simulink model "dual_thyristor_bridge_rectifier"  (R2025b)
settings: Solver=ode1be  StartTime=0.0  StopTime=simlength  FixedStep=tc  MaxStep=tc
values from neighbouring files (symbols this model uses):
  n1 = 35    [voltage_spectrum_analysis.m]
  omega_grid_emulator_nom = w_grid    (= 314.159265359)    [grid_emulator.m]
  vn_eta_pu = 0    [grid_emulator.m]
  vn_xi_pu = 0    [grid_emulator.m]
  vp_xi_pu = 1    [grid_emulator.m]
  w_grid = f_grid*2*pi    (= 314.159265359)    [grid_emulator.m]
undefined symbols (not defined in the file or in its folder): CSF_11, CSF_13, CSF_5, CSF_7, delta_fht1, Idc_traction_normalization_factor, ki_u_ctrl, kp_u_ctrl, Ld_fht1, LFu_dc, LSF_11, LSF_13, LSF_5, LSF_7, magnitude, n10, omega_fht1, pll_i1, pll_p, RLFu_dc, tc, Tcontrol_rect, ts_ctrl_rect, ugrid_factor, Vdc_traction_normalization_factor, Vgrid_phase_normalization_factor
libraries: fl_lib x299, nesl_utility x67, ee_lib x24, single_phase_transformer_lib x3, cstblocks x3
(part 5 of 6)

== system dual_thyristor_bridge_rectifier/dual_rectifier_bridge/pos_bridge/firing4 ==
  Capacitor1 : fl_lib/Electrical/Electrical Elements/Capacitor  Commented=on  c=100e-6 F  r=1e-6 Ohm  g=0 1/Ohm  i_specify=off  i_priority=None  i=0 A  i_nominal_specify=off  i_nominal_value=1  i_nominal_unit=A  v_specify=off  v_priority=None  v=0 V  v_nominal_specify=off  v_nominal_value=1  v_nominal_unit=V  vc_specify=off  vc_priority=High  vc=0 V  vc_nominal_specify=off  vc_nominal_value=1  vc_nominal_unit=V
  Capacitor2 : fl_lib/Electrical/Electrical Elements/Capacitor  Commented=on  c=100e-12 F  r=1e-6 Ohm  g=0 1/Ohm  i_specify=off  i_priority=None  i=0 A  i_nominal_specify=off  i_nominal_value=1  i_nominal_unit=A  v_specify=off  v_priority=None  v=0 V  v_nominal_specify=off  v_nominal_value=1  v_nominal_unit=V  vc_specify=off  vc_priority=High  vc=0 V  vc_nominal_specify=off  vc_nominal_value=1  vc_nominal_unit=V
  Controlled Voltage Source1 : fl_lib/Electrical/Electrical Sources/Controlled Voltage Source  Commented=on
  Controlled Voltage Source2 : fl_lib/Electrical/Electrical Sources/Controlled Voltage Source  Commented=on
  Diode : fl_lib/Electrical/Electrical Elements/Diode  Commented=on  Vf=0.6 V  Ron=0.3 Ohm  Goff=1e-8 1/Ohm  i_specify=off  i_priority=None  i=0 A  i_nominal_specify=off  i_nominal_value=1  i_nominal_unit=A  v_specify=off  v_priority=None  v=0 V  v_nominal_specify=off  v_nominal_value=1  v_nominal_unit=V
  Diode2 : fl_lib/Electrical/Electrical Elements/Diode  Commented=on  Vf=0.6 V  Ron=0.3 Ohm  Goff=1e-8 1/Ohm  i_specify=off  i_priority=None  i=0 A  i_nominal_specify=off  i_nominal_value=1  i_nominal_unit=A  v_specify=off  v_priority=None  v=0 V  v_nominal_specify=off  v_nominal_value=1  v_nominal_unit=V
  Diode3 : fl_lib/Electrical/Electrical Elements/Diode  Commented=on  Vf=0.6 V  Ron=0.3 Ohm  Goff=1e-8 1/Ohm  i_specify=off  i_priority=None  i=0 A  i_nominal_specify=off  i_nominal_value=1  i_nominal_unit=A  v_specify=off  v_priority=None  v=0 V  v_nominal_specify=off  v_nominal_value=1  v_nominal_unit=V
  Electrical Reference3 : fl_lib/Electrical/Electrical Elements/Electrical Reference  Commented=on
  Electrical Reference4 : fl_lib/Electrical/Electrical Elements/Electrical Reference  Commented=on
  Electrical Reference5 : fl_lib/Electrical/Electrical Elements/Electrical Reference  Commented=on
  "IGBT (Ideal, Switching)" : ee_lib/Semiconductors & Converters/IGBT (Ideal, Switching)  Commented=on  port_option=ee.enum.controlport.elec  Vf=0.8 V  Ron=0.001 Ohm  Goff=1e-5 1/Ohm  Vth=2 V  diode_param=1  diode_Vf=0.8 V  diode_Ron=0.001 Ohm  diode_Goff=1e-5 1/Ohm  diode_C=50e-9 F  diode_iRM=-235 A  diode_iF=300 A  diode_idot=-50 A/us  diode_trr_param=1  diode_trr_factor=3  diode_trr=15 us  diode_Qrr=1500 s*uA  ice_specify=off  ice_priority=None  ice=0 A  ice_nominal_specify=off  ice_nominal_value=1  ice_nominal_unit=A  vce_specify=off  vce_priority=None  vce=0 V  vce_nominal_specify=off  vce_nominal_value=1  vce_nominal_unit=V  vge_specify=off  vge_priority=None  vge=0 V  vge_nominal_specify=off  vge_nominal_value=1  vge_nominal_unit=V  thermal_loss_option=2  Von_data=[0, 1.1, 1.3, 1.45, 1.75, 2.25, 2.7; 0, 1, 1.15, 1.35, 1.7, 2.35, 3] V  Tj=[298.15, 398.15] K  Iout_data=[0, 10, 50, 100, 200, 400, 600] A  Eon_data=[0, .29, 1.43, 2.86, 5.71, 13.14, 22.86; 0, .57, 2.63, 5.14, 10.29, 20.57, 30.29] * 1e-3 J  Eoff_data=[0, .21, 1.07, 2.14, 4.29, 9.86, 17.14; 0, .43, 1.97, 3.86, 7.71, 15.43, 22.71] * 1e-3 J  Eon_data_3D=[zeros(2, 9, 3)] J  Eoff_data_3D=[zeros(2, 9, 3)] J  Tj_loss=[298.15, 398.15] K  Iout_data_loss=[0, .1, 1, 5, 10, 20, 40, 70, 100] A  tabulateWithVce=false  Vce_loss=[0, 150, 300] V  Eon_scalar=22.86e-3 J  Eoff_scalar=17.14e-3 J  Voff=300 V  Iout_scalar=600 A  useCurrentFromPreviousCycle=false  useVoltageFromPreviousCycle=false  diodeModelType=ee.enum.converters.diodeModelType.pwl  diodeTableType=ee.enum.diode.tableType.IfMat  diode_ReverseIVType=ee.enum.diode.diodeReverseIV.constant  diode_IfMat=[.07, .12, .19, 1.75, 4.24, 7.32, 11.2; .16, .3, .72, 2.14, 4.02, 6.35, 9.12] A  diode_VfMat=[.9, 1.15, 1.25, 1.5, 1.75, 2.17, 2.6, 2.85; .58, .68, .75, 1.1, 1.38, 1.77, 2.27, 2.7] V  diode_TjVec=[25, 125] degC  diode_VfVec=[.5, .7, .9, 1.3, 1.7, 2.1, 2.5] V  diode_IfVec=[.1, .2, .5, 1, 2, 4, 7, 10] A  diode_IrMat=[1e-06, 2e-06, 5e-06, 1e-05, 2.5e-05, 5e-05, .0001; 2e-06, 5e-06, 1e-05, 4e-05, 8e-05, .0002, .0005] A  diode_VrMat=[10, 100, 200, 250, 300, 325, 350; 10, 70, 160, 220, 270, 300, 320] V  diode_VrVec=[10, 20, 40, 50, 70, 80, 100] V  diode_IrVec=[1e-06, 2e-06, 5e-06, 1e-05, 2e-05, 5e-05, .0001] A  diode_Vr=-600 V  diode_Ls=150 nH  diode_Erec=0.03 J  diode_rec_loss_model=ee.enum.diode.reverseRecoveryModel.fixed  diode_ErecVal=0 J  diode_scaleWithIandV=true  diode_ErecMat=zeros(2, 3) J  diode_TjrecVec=[298.15, 398.15] K  diode_IfrecVec=[.1, 1, 10] A  diode_IrecVal=10 A  diode_VrecVal=10 V  diode_tFilter=1 / 1000 / 100 s  separateThermalPortForDiode=false  thermal_network_parameterization=ee.enum.thermalNetworkTopology.external  Rth=[.08, .5] K/W  Rth_Cauer=[.08, .1, .5] K/W  Rth_Foster=[.08, .14, .22, .16] K/W  thermal_mass_parameterization=ee.enum.thermalNetwork.timeconstant  thermal_mass=[.01, .5] J/K  thermal_mass_Cauer=[.01, .1, .5] J/K  thermal_mass_Foster=[.001, .005, .05, .5] J/K  thermal_time_constant=[.001, .2] s  thermal_time_constant_Cauer=[.001, .1, .2] s  thermal_time_constant_Foster=[7e-05, .0007, .01, .08] s  thermal_mass_initial_temperatures=[25, 25] degC  thermal_mass_initial_temperatures_Cauer=[25, 25, 25] degC  junction_thermal_mass=0.01 J/K  Tvec_initial_Foster=[25, 25, 25, 25] degC  RthDiode=[.03, .2] K/W  RthCauerDiode=[.03, .1, .2] K/W  RthFosterDiode=[.03, .2] K/W  thermalMassDiode=[3, 25] J/K  thermalMassCauerDiode=[3, 10, 25] J/K  thermalMassFosterDiode=[33, 50] J/K  thermalTauDiode=[.1, 5] s  thermalTauCauerDiode=[.1, 1, 5] s  thermalTauFosterDiode=[1, 10] s  thermalMassInitTempDiode=[25, 25] degC  thermalMassInitTempCauerDiode=[25, 25, 25] degC  junctionthermalMassDiode=0.1 J/K  TVecInitialFosterDiode=[25, 25, 25, 25] degC  no_thermal_network=0  IGBT_junction_temperature_specify=off  IGBT_junction_temperature_priority=None  IGBT_junction_temperature=25 degC  IGBT_junction_temperature_nominal_specify=off  IGBT_junction_temperature_nominal_value=1  IGBT_junction_temperature_nominal_unit=degC  diode_junction_temperature_specify=off  diode_junction_temperature_priority=None  diode_junction_temperature=25 degC  diode_junction_temperature_nominal_specify=off  diode_junction_temperature_nominal_value=1  diode_junction_temperature_nominal_unit=degC  Qj_specify=off  Qj_priority=None  Qj=0 W  Qj_nominal_specify=off  Qj_nominal_value=1  Qj_nominal_unit=W  accumulatedSwitchingLosses_specify=off  accumulatedSwitchingLosses_priority=None  accumulatedSwitchingLosses=0 J
      settings: InternalSimscapePortConfiguration="{\"Bottom\":[],\"Left\":[{\"id\":\"G_elec\",\"label\":\"\",\"type\":\"foundation.electrical.electrical\"}],\"Right\":[{\"id\":\"C\",\"label\":\"\",\"type\":\"foundation.electrical.electrical\"},{\"id\":\"E\",\"label\":\"\",\"type\":\"foundation.electrical.electrical\"}],\"Top\":[]}"
  Ideal Transformer : fl_lib/Electrical/Electrical Elements/Ideal Transformer  Commented=on  n=2  i1_specify=off  i1_priority=None  i1=0 A  i1_nominal_specify=off  i1_nominal_value=1  i1_nominal_unit=A  v1_specify=off  v1_priority=None  v1=0 V  v1_nominal_specify=off  v1_nominal_value=1  v1_nominal_unit=V  i2_specify=off  i2_priority=None  i2=0 A  i2_nominal_specify=off  i2_nominal_value=1  i2_nominal_unit=A  v2_specify=off  v2_priority=None  v2=0 V  v2_nominal_specify=off  v2_nominal_value=1  v2_nominal_unit=V
  PS Constant : fl_lib/Physical Signals/Sources/PS Constant  Commented=on  constant=48 V
  Resistor1 : fl_lib/Electrical/Electrical Elements/Resistor  Commented=on  R=470 Ohm  i_specify=off  i_priority=None  i=0 A  i_nominal_specify=off  i_nominal_value=1  i_nominal_unit=A  v_specify=off  v_priority=None  v=0 V  v_nominal_specify=off  v_nominal_value=1  v_nominal_unit=V
  Resistor3 : fl_lib/Electrical/Electrical Elements/Resistor  Commented=on  R=470 Ohm  i_specify=off  i_priority=None  i=0 A  i_nominal_specify=off  i_nominal_value=1  i_nominal_unit=A  v_specify=off  v_priority=None  v=0 V  v_nominal_specify=off  v_nominal_value=1  v_nominal_unit=V
  Resistor5 : fl_lib/Electrical/Electrical Elements/Resistor  Commented=on  R=100 Ohm  i_specify=off  i_priority=None  i=0 A  i_nominal_specify=off  i_nominal_value=1  i_nominal_unit=A  v_specify=off  v_priority=None  v=0 V  v_nominal_specify=off  v_nominal_value=1  v_nominal_unit=V
  Resistor6 : fl_lib/Electrical/Electrical Elements/Resistor  Commented=on  R=1e9 Ohm  i_specify=off  i_priority=None  i=0 A  i_nominal_specify=off  i_nominal_value=1  i_nominal_unit=A  v_specify=off  v_priority=None  v=0 V  v_nominal_specify=off  v_nominal_value=1  v_nominal_unit=V
  Voltage Sensor : fl_lib/Electrical/Electrical Sensors/Voltage Sensor  Commented=on
  oscillator : Subsystem  Commented=on
  gin : PMIOPort  Side=Left
  g+ : PMIOPort  Port=2  Side=Right
  connections:
  gin/RConn1 -- g+/RConn1
  Resistor3/LConn1 -- Controlled Voltage Source1/LConn1
  Electrical Reference5/LConn1 -- Capacitor1/RConn1
  Capacitor1/LConn1 -- Resistor3/RConn1 -- Diode3/LConn1
  "IGBT (Ideal, Switching)"/RConn1 -- Diode3/RConn1
  Resistor6/RConn1 -- Electrical Reference3/LConn1
  PS Constant/RConn1 -- Controlled Voltage Source1/RConn1
  Capacitor2/LConn1 -- Voltage Sensor/LConn1 -- Resistor5/LConn1 -- Diode2/RConn1
  Resistor5/RConn1 -- Resistor6/LConn1 -- Ideal Transformer/RConn2 -- Voltage Sensor/RConn2 -- Capacitor2/RConn1
  Ideal Transformer/RConn1 -- Diode2/LConn1
  Diode/RConn1 -- Ideal Transformer/LConn1 -- "IGBT (Ideal, Switching)"/RConn2 -- Controlled Voltage Source1/RConn2 -- Controlled Voltage Source2/RConn2
  Controlled Voltage Source2/LConn1 -- Resistor1/LConn1
  Ideal Transformer/LConn2 -- Diode/LConn1 -- Electrical Reference4/LConn1
  "IGBT (Ideal, Switching)"/LConn1 -- Resistor1/RConn1

== system dual_thyristor_bridge_rectifier/dual_rectifier_bridge/pos_bridge/firing5 ==
  Capacitor1 : fl_lib/Electrical/Electrical Elements/Capacitor  Commented=on  c=100e-6 F  r=1e-6 Ohm  g=0 1/Ohm  i_specify=off  i_priority=None  i=0 A  i_nominal_specify=off  i_nominal_value=1  i_nominal_unit=A  v_specify=off  v_priority=None  v=0 V  v_nominal_specify=off  v_nominal_value=1  v_nominal_unit=V  vc_specify=off  vc_priority=High  vc=0 V  vc_nominal_specify=off  vc_nominal_value=1  vc_nominal_unit=V
  Capacitor2 : fl_lib/Electrical/Electrical Elements/Capacitor  Commented=on  c=100e-12 F  r=1e-6 Ohm  g=0 1/Ohm  i_specify=off  i_priority=None  i=0 A  i_nominal_specify=off  i_nominal_value=1  i_nominal_unit=A  v_specify=off  v_priority=None  v=0 V  v_nominal_specify=off  v_nominal_value=1  v_nominal_unit=V  vc_specify=off  vc_priority=High  vc=0 V  vc_nominal_specify=off  vc_nominal_value=1  vc_nominal_unit=V
  Controlled Voltage Source1 : fl_lib/Electrical/Electrical Sources/Controlled Voltage Source  Commented=on
  Controlled Voltage Source2 : fl_lib/Electrical/Electrical Sources/Controlled Voltage Source  Commented=on
  Diode : fl_lib/Electrical/Electrical Elements/Diode  Commented=on  Vf=0.6 V  Ron=0.3 Ohm  Goff=1e-8 1/Ohm  i_specify=off  i_priority=None  i=0 A  i_nominal_specify=off  i_nominal_value=1  i_nominal_unit=A  v_specify=off  v_priority=None  v=0 V  v_nominal_specify=off  v_nominal_value=1  v_nominal_unit=V
  Diode2 : fl_lib/Electrical/Electrical Elements/Diode  Commented=on  Vf=0.6 V  Ron=0.3 Ohm  Goff=1e-8 1/Ohm  i_specify=off  i_priority=None  i=0 A  i_nominal_specify=off  i_nominal_value=1  i_nominal_unit=A  v_specify=off  v_priority=None  v=0 V  v_nominal_specify=off  v_nominal_value=1  v_nominal_unit=V
  Diode3 : fl_lib/Electrical/Electrical Elements/Diode  Commented=on  Vf=0.6 V  Ron=0.3 Ohm  Goff=1e-8 1/Ohm  i_specify=off  i_priority=None  i=0 A  i_nominal_specify=off  i_nominal_value=1  i_nominal_unit=A  v_specify=off  v_priority=None  v=0 V  v_nominal_specify=off  v_nominal_value=1  v_nominal_unit=V
  Electrical Reference3 : fl_lib/Electrical/Electrical Elements/Electrical Reference  Commented=on
  Electrical Reference4 : fl_lib/Electrical/Electrical Elements/Electrical Reference  Commented=on
  Electrical Reference5 : fl_lib/Electrical/Electrical Elements/Electrical Reference  Commented=on
  "IGBT (Ideal, Switching)" : ee_lib/Semiconductors & Converters/IGBT (Ideal, Switching)  Commented=on  port_option=ee.enum.controlport.elec  Vf=0.8 V  Ron=0.001 Ohm  Goff=1e-5 1/Ohm  Vth=2 V  diode_param=1  diode_Vf=0.8 V  diode_Ron=0.001 Ohm  diode_Goff=1e-5 1/Ohm  diode_C=50e-9 F  diode_iRM=-235 A  diode_iF=300 A  diode_idot=-50 A/us  diode_trr_param=1  diode_trr_factor=3  diode_trr=15 us  diode_Qrr=1500 s*uA  ice_specify=off  ice_priority=None  ice=0 A  ice_nominal_specify=off  ice_nominal_value=1  ice_nominal_unit=A  vce_specify=off  vce_priority=None  vce=0 V  vce_nominal_specify=off  vce_nominal_value=1  vce_nominal_unit=V  vge_specify=off  vge_priority=None  vge=0 V  vge_nominal_specify=off  vge_nominal_value=1  vge_nominal_unit=V  thermal_loss_option=2  Von_data=[0, 1.1, 1.3, 1.45, 1.75, 2.25, 2.7; 0, 1, 1.15, 1.35, 1.7, 2.35, 3] V  Tj=[298.15, 398.15] K  Iout_data=[0, 10, 50, 100, 200, 400, 600] A  Eon_data=[0, .29, 1.43, 2.86, 5.71, 13.14, 22.86; 0, .57, 2.63, 5.14, 10.29, 20.57, 30.29] * 1e-3 J  Eoff_data=[0, .21, 1.07, 2.14, 4.29, 9.86, 17.14; 0, .43, 1.97, 3.86, 7.71, 15.43, 22.71] * 1e-3 J  Eon_data_3D=[zeros(2, 9, 3)] J  Eoff_data_3D=[zeros(2, 9, 3)] J  Tj_loss=[298.15, 398.15] K  Iout_data_loss=[0, .1, 1, 5, 10, 20, 40, 70, 100] A  tabulateWithVce=false  Vce_loss=[0, 150, 300] V  Eon_scalar=22.86e-3 J  Eoff_scalar=17.14e-3 J  Voff=300 V  Iout_scalar=600 A  useCurrentFromPreviousCycle=false  useVoltageFromPreviousCycle=false  diodeModelType=ee.enum.converters.diodeModelType.pwl  diodeTableType=ee.enum.diode.tableType.IfMat  diode_ReverseIVType=ee.enum.diode.diodeReverseIV.constant  diode_IfMat=[.07, .12, .19, 1.75, 4.24, 7.32, 11.2; .16, .3, .72, 2.14, 4.02, 6.35, 9.12] A  diode_VfMat=[.9, 1.15, 1.25, 1.5, 1.75, 2.17, 2.6, 2.85; .58, .68, .75, 1.1, 1.38, 1.77, 2.27, 2.7] V  diode_TjVec=[25, 125] degC  diode_VfVec=[.5, .7, .9, 1.3, 1.7, 2.1, 2.5] V  diode_IfVec=[.1, .2, .5, 1, 2, 4, 7, 10] A  diode_IrMat=[1e-06, 2e-06, 5e-06, 1e-05, 2.5e-05, 5e-05, .0001; 2e-06, 5e-06, 1e-05, 4e-05, 8e-05, .0002, .0005] A  diode_VrMat=[10, 100, 200, 250, 300, 325, 350; 10, 70, 160, 220, 270, 300, 320] V  diode_VrVec=[10, 20, 40, 50, 70, 80, 100] V  diode_IrVec=[1e-06, 2e-06, 5e-06, 1e-05, 2e-05, 5e-05, .0001] A  diode_Vr=-600 V  diode_Ls=150 nH  diode_Erec=0.03 J  diode_rec_loss_model=ee.enum.diode.reverseRecoveryModel.fixed  diode_ErecVal=0 J  diode_scaleWithIandV=true  diode_ErecMat=zeros(2, 3) J  diode_TjrecVec=[298.15, 398.15] K  diode_IfrecVec=[.1, 1, 10] A  diode_IrecVal=10 A  diode_VrecVal=10 V  diode_tFilter=1 / 1000 / 100 s  separateThermalPortForDiode=false  thermal_network_parameterization=ee.enum.thermalNetworkTopology.external  Rth=[.08, .5] K/W  Rth_Cauer=[.08, .1, .5] K/W  Rth_Foster=[.08, .14, .22, .16] K/W  thermal_mass_parameterization=ee.enum.thermalNetwork.timeconstant  thermal_mass=[.01, .5] J/K  thermal_mass_Cauer=[.01, .1, .5] J/K  thermal_mass_Foster=[.001, .005, .05, .5] J/K  thermal_time_constant=[.001, .2] s  thermal_time_constant_Cauer=[.001, .1, .2] s  thermal_time_constant_Foster=[7e-05, .0007, .01, .08] s  thermal_mass_initial_temperatures=[25, 25] degC  thermal_mass_initial_temperatures_Cauer=[25, 25, 25] degC  junction_thermal_mass=0.01 J/K  Tvec_initial_Foster=[25, 25, 25, 25] degC  RthDiode=[.03, .2] K/W  RthCauerDiode=[.03, .1, .2] K/W  RthFosterDiode=[.03, .2] K/W  thermalMassDiode=[3, 25] J/K  thermalMassCauerDiode=[3, 10, 25] J/K  thermalMassFosterDiode=[33, 50] J/K  thermalTauDiode=[.1, 5] s  thermalTauCauerDiode=[.1, 1, 5] s  thermalTauFosterDiode=[1, 10] s  thermalMassInitTempDiode=[25, 25] degC  thermalMassInitTempCauerDiode=[25, 25, 25] degC  junctionthermalMassDiode=0.1 J/K  TVecInitialFosterDiode=[25, 25, 25, 25] degC  no_thermal_network=0  IGBT_junction_temperature_specify=off  IGBT_junction_temperature_priority=None  IGBT_junction_temperature=25 degC  IGBT_junction_temperature_nominal_specify=off  IGBT_junction_temperature_nominal_value=1  IGBT_junction_temperature_nominal_unit=degC  diode_junction_temperature_specify=off  diode_junction_temperature_priority=None  diode_junction_temperature=25 degC  diode_junction_temperature_nominal_specify=off  diode_junction_temperature_nominal_value=1  diode_junction_temperature_nominal_unit=degC  Qj_specify=off  Qj_priority=None  Qj=0 W  Qj_nominal_specify=off  Qj_nominal_value=1  Qj_nominal_unit=W  accumulatedSwitchingLosses_specify=off  accumulatedSwitchingLosses_priority=None  accumulatedSwitchingLosses=0 J
      settings: InternalSimscapePortConfiguration="{\"Bottom\":[],\"Left\":[{\"id\":\"G_elec\",\"label\":\"\",\"type\":\"foundation.electrical.electrical\"}],\"Right\":[{\"id\":\"C\",\"label\":\"\",\"type\":\"foundation.electrical.electrical\"},{\"id\":\"E\",\"label\":\"\",\"type\":\"foundation.electrical.electrical\"}],\"Top\":[]}"
  Ideal Transformer : fl_lib/Electrical/Electrical Elements/Ideal Transformer  Commented=on  n=2  i1_specify=off  i1_priority=None  i1=0 A  i1_nominal_specify=off  i1_nominal_value=1  i1_nominal_unit=A  v1_specify=off  v1_priority=None  v1=0 V  v1_nominal_specify=off  v1_nominal_value=1  v1_nominal_unit=V  i2_specify=off  i2_priority=None  i2=0 A  i2_nominal_specify=off  i2_nominal_value=1  i2_nominal_unit=A  v2_specify=off  v2_priority=None  v2=0 V  v2_nominal_specify=off  v2_nominal_value=1  v2_nominal_unit=V
  PS Constant : fl_lib/Physical Signals/Sources/PS Constant  Commented=on  constant=48 V
  Resistor1 : fl_lib/Electrical/Electrical Elements/Resistor  Commented=on  R=470 Ohm  i_specify=off  i_priority=None  i=0 A  i_nominal_specify=off  i_nominal_value=1  i_nominal_unit=A  v_specify=off  v_priority=None  v=0 V  v_nominal_specify=off  v_nominal_value=1  v_nominal_unit=V
  Resistor3 : fl_lib/Electrical/Electrical Elements/Resistor  Commented=on  R=470 Ohm  i_specify=off  i_priority=None  i=0 A  i_nominal_specify=off  i_nominal_value=1  i_nominal_unit=A  v_specify=off  v_priority=None  v=0 V  v_nominal_specify=off  v_nominal_value=1  v_nominal_unit=V
  Resistor5 : fl_lib/Electrical/Electrical Elements/Resistor  Commented=on  R=100 Ohm  i_specify=off  i_priority=None  i=0 A  i_nominal_specify=off  i_nominal_value=1  i_nominal_unit=A  v_specify=off  v_priority=None  v=0 V  v_nominal_specify=off  v_nominal_value=1  v_nominal_unit=V
  Resistor6 : fl_lib/Electrical/Electrical Elements/Resistor  Commented=on  R=1e9 Ohm  i_specify=off  i_priority=None  i=0 A  i_nominal_specify=off  i_nominal_value=1  i_nominal_unit=A  v_specify=off  v_priority=None  v=0 V  v_nominal_specify=off  v_nominal_value=1  v_nominal_unit=V
  Voltage Sensor : fl_lib/Electrical/Electrical Sensors/Voltage Sensor  Commented=on
  oscillator : Subsystem  Commented=on
  gin : PMIOPort  Side=Left
  g+ : PMIOPort  Port=2  Side=Right
  connections:
  gin/RConn1 -- g+/RConn1
  "IGBT (Ideal, Switching)"/LConn1 -- Resistor1/RConn1
  Electrical Reference4/LConn1 -- Diode/LConn1 -- Ideal Transformer/LConn2
  Controlled Voltage Source2/LConn1 -- Resistor1/LConn1
  Controlled Voltage Source2/RConn2 -- Controlled Voltage Source1/RConn2 -- "IGBT (Ideal, Switching)"/RConn2 -- Ideal Transformer/LConn1 -- Diode/RConn1
  Ideal Transformer/RConn1 -- Diode2/LConn1
  Capacitor2/RConn1 -- Voltage Sensor/RConn2 -- Ideal Transformer/RConn2 -- Resistor6/LConn1 -- Resistor5/RConn1
  Diode2/RConn1 -- Resistor5/LConn1 -- Voltage Sensor/LConn1 -- Capacitor2/LConn1
  PS Constant/RConn1 -- Controlled Voltage Source1/RConn1
  Resistor6/RConn1 -- Electrical Reference3/LConn1
  "IGBT (Ideal, Switching)"/RConn1 -- Diode3/RConn1
  Diode3/LConn1 -- Resistor3/RConn1 -- Capacitor1/LConn1
  Electrical Reference5/LConn1 -- Capacitor1/RConn1
  Resistor3/LConn1 -- Controlled Voltage Source1/LConn1

== system dual_thyristor_bridge_rectifier/dual_rectifier_bridge/pos_bridge/firing6 ==
  Capacitor1 : fl_lib/Electrical/Electrical Elements/Capacitor  Commented=on  c=100e-6 F  r=1e-6 Ohm  g=0 1/Ohm  i_specify=off  i_priority=None  i=0 A  i_nominal_specify=off  i_nominal_value=1  i_nominal_unit=A  v_specify=off  v_priority=None  v=0 V  v_nominal_specify=off  v_nominal_value=1  v_nominal_unit=V  vc_specify=off  vc_priority=High  vc=0 V  vc_nominal_specify=off  vc_nominal_value=1  vc_nominal_unit=V
  Capacitor2 : fl_lib/Electrical/Electrical Elements/Capacitor  Commented=on  c=100e-12 F  r=1e-6 Ohm  g=0 1/Ohm  i_specify=off  i_priority=None  i=0 A  i_nominal_specify=off  i_nominal_value=1  i_nominal_unit=A  v_specify=off  v_priority=None  v=0 V  v_nominal_specify=off  v_nominal_value=1  v_nominal_unit=V  vc_specify=off  vc_priority=High  vc=0 V  vc_nominal_specify=off  vc_nominal_value=1  vc_nominal_unit=V
  Controlled Voltage Source1 : fl_lib/Electrical/Electrical Sources/Controlled Voltage Source  Commented=on
  Controlled Voltage Source2 : fl_lib/Electrical/Electrical Sources/Controlled Voltage Source  Commented=on
  Diode : fl_lib/Electrical/Electrical Elements/Diode  Commented=on  Vf=0.6 V  Ron=0.3 Ohm  Goff=1e-8 1/Ohm  i_specify=off  i_priority=None  i=0 A  i_nominal_specify=off  i_nominal_value=1  i_nominal_unit=A  v_specify=off  v_priority=None  v=0 V  v_nominal_specify=off  v_nominal_value=1  v_nominal_unit=V
  Diode2 : fl_lib/Electrical/Electrical Elements/Diode  Commented=on  Vf=0.6 V  Ron=0.3 Ohm  Goff=1e-8 1/Ohm  i_specify=off  i_priority=None  i=0 A  i_nominal_specify=off  i_nominal_value=1  i_nominal_unit=A  v_specify=off  v_priority=None  v=0 V  v_nominal_specify=off  v_nominal_value=1  v_nominal_unit=V
  Diode3 : fl_lib/Electrical/Electrical Elements/Diode  Commented=on  Vf=0.6 V  Ron=0.3 Ohm  Goff=1e-8 1/Ohm  i_specify=off  i_priority=None  i=0 A  i_nominal_specify=off  i_nominal_value=1  i_nominal_unit=A  v_specify=off  v_priority=None  v=0 V  v_nominal_specify=off  v_nominal_value=1  v_nominal_unit=V
  Electrical Reference3 : fl_lib/Electrical/Electrical Elements/Electrical Reference  Commented=on
  Electrical Reference4 : fl_lib/Electrical/Electrical Elements/Electrical Reference  Commented=on
  Electrical Reference5 : fl_lib/Electrical/Electrical Elements/Electrical Reference  Commented=on
  "IGBT (Ideal, Switching)" : ee_lib/Semiconductors & Converters/IGBT (Ideal, Switching)  Commented=on  port_option=ee.enum.controlport.elec  Vf=0.8 V  Ron=0.001 Ohm  Goff=1e-5 1/Ohm  Vth=2 V  diode_param=1  diode_Vf=0.8 V  diode_Ron=0.001 Ohm  diode_Goff=1e-5 1/Ohm  diode_C=50e-9 F  diode_iRM=-235 A  diode_iF=300 A  diode_idot=-50 A/us  diode_trr_param=1  diode_trr_factor=3  diode_trr=15 us  diode_Qrr=1500 s*uA  ice_specify=off  ice_priority=None  ice=0 A  ice_nominal_specify=off  ice_nominal_value=1  ice_nominal_unit=A  vce_specify=off  vce_priority=None  vce=0 V  vce_nominal_specify=off  vce_nominal_value=1  vce_nominal_unit=V  vge_specify=off  vge_priority=None  vge=0 V  vge_nominal_specify=off  vge_nominal_value=1  vge_nominal_unit=V  thermal_loss_option=2  Von_data=[0, 1.1, 1.3, 1.45, 1.75, 2.25, 2.7; 0, 1, 1.15, 1.35, 1.7, 2.35, 3] V  Tj=[298.15, 398.15] K  Iout_data=[0, 10, 50, 100, 200, 400, 600] A  Eon_data=[0, .29, 1.43, 2.86, 5.71, 13.14, 22.86; 0, .57, 2.63, 5.14, 10.29, 20.57, 30.29] * 1e-3 J  Eoff_data=[0, .21, 1.07, 2.14, 4.29, 9.86, 17.14; 0, .43, 1.97, 3.86, 7.71, 15.43, 22.71] * 1e-3 J  Eon_data_3D=[zeros(2, 9, 3)] J  Eoff_data_3D=[zeros(2, 9, 3)] J  Tj_loss=[298.15, 398.15] K  Iout_data_loss=[0, .1, 1, 5, 10, 20, 40, 70, 100] A  tabulateWithVce=false  Vce_loss=[0, 150, 300] V  Eon_scalar=22.86e-3 J  Eoff_scalar=17.14e-3 J  Voff=300 V  Iout_scalar=600 A  useCurrentFromPreviousCycle=false  useVoltageFromPreviousCycle=false  diodeModelType=ee.enum.converters.diodeModelType.pwl  diodeTableType=ee.enum.diode.tableType.IfMat  diode_ReverseIVType=ee.enum.diode.diodeReverseIV.constant  diode_IfMat=[.07, .12, .19, 1.75, 4.24, 7.32, 11.2; .16, .3, .72, 2.14, 4.02, 6.35, 9.12] A  diode_VfMat=[.9, 1.15, 1.25, 1.5, 1.75, 2.17, 2.6, 2.85; .58, .68, .75, 1.1, 1.38, 1.77, 2.27, 2.7] V  diode_TjVec=[25, 125] degC  diode_VfVec=[.5, .7, .9, 1.3, 1.7, 2.1, 2.5] V  diode_IfVec=[.1, .2, .5, 1, 2, 4, 7, 10] A  diode_IrMat=[1e-06, 2e-06, 5e-06, 1e-05, 2.5e-05, 5e-05, .0001; 2e-06, 5e-06, 1e-05, 4e-05, 8e-05, .0002, .0005] A  diode_VrMat=[10, 100, 200, 250, 300, 325, 350; 10, 70, 160, 220, 270, 300, 320] V  diode_VrVec=[10, 20, 40, 50, 70, 80, 100] V  diode_IrVec=[1e-06, 2e-06, 5e-06, 1e-05, 2e-05, 5e-05, .0001] A  diode_Vr=-600 V  diode_Ls=150 nH  diode_Erec=0.03 J  diode_rec_loss_model=ee.enum.diode.reverseRecoveryModel.fixed  diode_ErecVal=0 J  diode_scaleWithIandV=true  diode_ErecMat=zeros(2, 3) J  diode_TjrecVec=[298.15, 398.15] K  diode_IfrecVec=[.1, 1, 10] A  diode_IrecVal=10 A  diode_VrecVal=10 V  diode_tFilter=1 / 1000 / 100 s  separateThermalPortForDiode=false  thermal_network_parameterization=ee.enum.thermalNetworkTopology.external  Rth=[.08, .5] K/W  Rth_Cauer=[.08, .1, .5] K/W  Rth_Foster=[.08, .14, .22, .16] K/W  thermal_mass_parameterization=ee.enum.thermalNetwork.timeconstant  thermal_mass=[.01, .5] J/K  thermal_mass_Cauer=[.01, .1, .5] J/K  thermal_mass_Foster=[.001, .005, .05, .5] J/K  thermal_time_constant=[.001, .2] s  thermal_time_constant_Cauer=[.001, .1, .2] s  thermal_time_constant_Foster=[7e-05, .0007, .01, .08] s  thermal_mass_initial_temperatures=[25, 25] degC  thermal_mass_initial_temperatures_Cauer=[25, 25, 25] degC  junction_thermal_mass=0.01 J/K  Tvec_initial_Foster=[25, 25, 25, 25] degC  RthDiode=[.03, .2] K/W  RthCauerDiode=[.03, .1, .2] K/W  RthFosterDiode=[.03, .2] K/W  thermalMassDiode=[3, 25] J/K  thermalMassCauerDiode=[3, 10, 25] J/K  thermalMassFosterDiode=[33, 50] J/K  thermalTauDiode=[.1, 5] s  thermalTauCauerDiode=[.1, 1, 5] s  thermalTauFosterDiode=[1, 10] s  thermalMassInitTempDiode=[25, 25] degC  thermalMassInitTempCauerDiode=[25, 25, 25] degC  junctionthermalMassDiode=0.1 J/K  TVecInitialFosterDiode=[25, 25, 25, 25] degC  no_thermal_network=0  IGBT_junction_temperature_specify=off  IGBT_junction_temperature_priority=None  IGBT_junction_temperature=25 degC  IGBT_junction_temperature_nominal_specify=off  IGBT_junction_temperature_nominal_value=1  IGBT_junction_temperature_nominal_unit=degC  diode_junction_temperature_specify=off  diode_junction_temperature_priority=None  diode_junction_temperature=25 degC  diode_junction_temperature_nominal_specify=off  diode_junction_temperature_nominal_value=1  diode_junction_temperature_nominal_unit=degC  Qj_specify=off  Qj_priority=None  Qj=0 W  Qj_nominal_specify=off  Qj_nominal_value=1  Qj_nominal_unit=W  accumulatedSwitchingLosses_specify=off  accumulatedSwitchingLosses_priority=None  accumulatedSwitchingLosses=0 J
      settings: InternalSimscapePortConfiguration="{\"Bottom\":[],\"Left\":[{\"id\":\"G_elec\",\"label\":\"\",\"type\":\"foundation.electrical.electrical\"}],\"Right\":[{\"id\":\"C\",\"label\":\"\",\"type\":\"foundation.electrical.electrical\"},{\"id\":\"E\",\"label\":\"\",\"type\":\"foundation.electrical.electrical\"}],\"Top\":[]}"
  Ideal Transformer : fl_lib/Electrical/Electrical Elements/Ideal Transformer  Commented=on  n=2  i1_specify=off  i1_priority=None  i1=0 A  i1_nominal_specify=off  i1_nominal_value=1  i1_nominal_unit=A  v1_specify=off  v1_priority=None  v1=0 V  v1_nominal_specify=off  v1_nominal_value=1  v1_nominal_unit=V  i2_specify=off  i2_priority=None  i2=0 A  i2_nominal_specify=off  i2_nominal_value=1  i2_nominal_unit=A  v2_specify=off  v2_priority=None  v2=0 V  v2_nominal_specify=off  v2_nominal_value=1  v2_nominal_unit=V
  PS Constant : fl_lib/Physical Signals/Sources/PS Constant  Commented=on  constant=48 V
  Resistor1 : fl_lib/Electrical/Electrical Elements/Resistor  Commented=on  R=470 Ohm  i_specify=off  i_priority=None  i=0 A  i_nominal_specify=off  i_nominal_value=1  i_nominal_unit=A  v_specify=off  v_priority=None  v=0 V  v_nominal_specify=off  v_nominal_value=1  v_nominal_unit=V
  Resistor3 : fl_lib/Electrical/Electrical Elements/Resistor  Commented=on  R=470 Ohm  i_specify=off  i_priority=None  i=0 A  i_nominal_specify=off  i_nominal_value=1  i_nominal_unit=A  v_specify=off  v_priority=None  v=0 V  v_nominal_specify=off  v_nominal_value=1  v_nominal_unit=V
  Resistor5 : fl_lib/Electrical/Electrical Elements/Resistor  Commented=on  R=100 Ohm  i_specify=off  i_priority=None  i=0 A  i_nominal_specify=off  i_nominal_value=1  i_nominal_unit=A  v_specify=off  v_priority=None  v=0 V  v_nominal_specify=off  v_nominal_value=1  v_nominal_unit=V
  Resistor6 : fl_lib/Electrical/Electrical Elements/Resistor  Commented=on  R=1e9 Ohm  i_specify=off  i_priority=None  i=0 A  i_nominal_specify=off  i_nominal_value=1  i_nominal_unit=A  v_specify=off  v_priority=None  v=0 V  v_nominal_specify=off  v_nominal_value=1  v_nominal_unit=V
  Voltage Sensor : fl_lib/Electrical/Electrical Sensors/Voltage Sensor  Commented=on
  oscillator : Subsystem  Commented=on
  gin : PMIOPort  Side=Left
  g+ : PMIOPort  Port=2  Side=Right
  connections:
  gin/RConn1 -- g+/RConn1
  Resistor3/LConn1 -- Controlled Voltage Source1/LConn1
  Electrical Reference5/LConn1 -- Capacitor1/RConn1
  Capacitor1/LConn1 -- Resistor3/RConn1 -- Diode3/LConn1
  "IGBT (Ideal, Switching)"/RConn1 -- Diode3/RConn1
  Resistor6/RConn1 -- Electrical Reference3/LConn1
  PS Constant/RConn1 -- Controlled Voltage Source1/RConn1
  Capacitor2/LConn1 -- Voltage Sensor/LConn1 -- Resistor5/LConn1 -- Diode2/RConn1
  Resistor5/RConn1 -- Resistor6/LConn1 -- Ideal Transformer/RConn2 -- Voltage Sensor/RConn2 -- Capacitor2/RConn1
  Ideal Transformer/RConn1 -- Diode2/LConn1
  Diode/RConn1 -- Ideal Transformer/LConn1 -- "IGBT (Ideal, Switching)"/RConn2 -- Controlled Voltage Source1/RConn2 -- Controlled Voltage Source2/RConn2
  Controlled Voltage Source2/LConn1 -- Resistor1/LConn1
  Ideal Transformer/LConn2 -- Diode/LConn1 -- Electrical Reference4/LConn1
  "IGBT (Ideal, Switching)"/LConn1 -- Resistor1/RConn1

== system dual_thyristor_bridge_rectifier/grid/grid_emulator/3ph_Dyg ==
  Electrical Reference1 : fl_lib/Electrical/Electrical Elements/Electrical Reference
  ph1 : single_phase_transformer_lib/single phase transformer  Lm=Lmu2_trafo H  n1=50*sqrt(3)  n2=50  Rd1=0 Ohm  Rd2=Rd2_trafo Ohm  Ld1=0 H  Ld2=Ld2_trafo H  Rfe=Rm2_trafo Ohm  phi_specify=off  phi_priority=None  phi=0 V*s  phi_nominal_specify=off  phi_nominal_value=1  phi_nominal_unit=V*s  i1_specify=off  i1_priority=None  i1=0 A  i1_nominal_specify=off  i1_nominal_value=1  i1_nominal_unit=A  i2_specify=off  i2_priority=None  i2=0 A  i2_nominal_specify=off  i2_nominal_value=1  i2_nominal_unit=A  ife_specify=off  ife_priority=None  ife=0 A  ife_nominal_specify=off  ife_nominal_value=1  ife_nominal_unit=A  u1_specify=off  u1_priority=None  u1=0 V  u1_nominal_specify=off  u1_nominal_value=1  u1_nominal_unit=V  u2_specify=off  u2_priority=None  u2=0 V  u2_nominal_specify=off  u2_nominal_value=1  u2_nominal_unit=V
      settings: InternalSimscapePortConfiguration="{\"Bottom\":[],\"Left\":[{\"id\":\"u1_p\",\"label\":\"u1(+)\",\"type\":\"foundation.electrical.electrical\"},{\"id\":\"u1_n\",\"label\":\"u1(-)\",\"type\":\"foundation.electrical.electrical\"}],\"Right\":[{\"id\":\"u2_p\",\"label\":\"u2(+)\",\"type\":\"foundation.electrical.electrical\"},{\"id\":\"u2_n\",\"label\":\"u2(-)\",\"type\":\"foundation.electrical.electrical\"}],\"Top\":[]}"
  ph2 : single_phase_transformer_lib/single phase transformer  Lm=Lmu2_trafo H  n1=50*sqrt(3)  n2=50  Rd1=0 Ohm  Rd2=Rd2_trafo Ohm  Ld1=0 H  Ld2=Ld2_trafo H  Rfe=Rm2_trafo Ohm  phi_specify=off  phi_priority=None  phi=0 V*s  phi_nominal_specify=off  phi_nominal_value=1  phi_nominal_unit=V*s  i1_specify=off  i1_priority=None  i1=0 A  i1_nominal_specify=off  i1_nominal_value=1  i1_nominal_unit=A  i2_specify=off  i2_priority=None  i2=0 A  i2_nominal_specify=off  i2_nominal_value=1  i2_nominal_unit=A  ife_specify=off  ife_priority=None  ife=0 A  ife_nominal_specify=off  ife_nominal_value=1  ife_nominal_unit=A  u1_specify=off  u1_priority=None  u1=0 V  u1_nominal_specify=off  u1_nominal_value=1  u1_nominal_unit=V  u2_specify=off  u2_priority=None  u2=0 V  u2_nominal_specify=off  u2_nominal_value=1  u2_nominal_unit=V
      settings: InternalSimscapePortConfiguration="{\"Bottom\":[],\"Left\":[{\"id\":\"u1_p\",\"label\":\"u1(+)\",\"type\":\"foundation.electrical.electrical\"},{\"id\":\"u1_n\",\"label\":\"u1(-)\",\"type\":\"foundation.electrical.electrical\"}],\"Right\":[{\"id\":\"u2_p\",\"label\":\"u2(+)\",\"type\":\"foundation.electrical.electrical\"},{\"id\":\"u2_n\",\"label\":\"u2(-)\",\"type\":\"foundation.electrical.electrical\"}],\"Top\":[]}"
  ph3 : single_phase_transformer_lib/single phase transformer  Lm=Lmu2_trafo H  n1=50*sqrt(3)  n2=50  Rd1=0 Ohm  Rd2=Rd2_trafo Ohm  Ld1=0 H  Ld2=Ld2_trafo H  Rfe=Rm2_trafo Ohm  phi_specify=off  phi_priority=None  phi=0 V*s  phi_nominal_specify=off  phi_nominal_value=1  phi_nominal_unit=V*s  i1_specify=off  i1_priority=None  i1=0 A  i1_nominal_specify=off  i1_nominal_value=1  i1_nominal_unit=A  i2_specify=off  i2_priority=None  i2=0 A  i2_nominal_specify=off  i2_nominal_value=1  i2_nominal_unit=A  ife_specify=off  ife_priority=None  ife=0 A  ife_nominal_specify=off  ife_nominal_value=1  ife_nominal_unit=A  u1_specify=off  u1_priority=None  u1=0 V  u1_nominal_specify=off  u1_nominal_value=1  u1_nominal_unit=V  u2_specify=off  u2_priority=None  u2=0 V  u2_nominal_specify=off  u2_nominal_value=1  u2_nominal_unit=V
      settings: InternalSimscapePortConfiguration="{\"Bottom\":[],\"Left\":[{\"id\":\"u1_p\",\"label\":\"u1(+)\",\"type\":\"foundation.electrical.electrical\"},{\"id\":\"u1_n\",\"label\":\"u1(-)\",\"type\":\"foundation.electrical.electrical\"}],\"Right\":[{\"id\":\"u2_p\",\"label\":\"u2(+)\",\"type\":\"foundation.electrical.electrical\"},{\"id\":\"u2_n\",\"label\":\"u2(-)\",\"type\":\"foundation.electrical.electrical\"}],\"Top\":[]}"
  ua : PMIOPort  Side=Right
  ub : PMIOPort  Port=2  Side=Right
  uc : PMIOPort  Port=3  Side=Right
  Ua : PMIOPort  Port=4  Side=Left
  Ub : PMIOPort  Port=5  Side=Left
  Uc : PMIOPort  Port=6  Side=Left
  connections:
  Electrical Reference1/LConn1 -- ph3/RConn2 -- ph2/RConn2 -- ph1/RConn2
  ph3/RConn1 -- uc/RConn1
  ph1/LConn1 -- ph3/LConn2 -- Ua/RConn1
  ph1/RConn1 -- ua/RConn1
  ph2/RConn1 -- ub/RConn1
  ph1/LConn2 -- ph2/LConn1 -- Ub/RConn1
  Uc/RConn1 -- ph3/LConn1 -- ph2/LConn2

== system dual_thyristor_bridge_rectifier/grid/grid_emulator/grid_emulator ==
  phase_gen : Subsystem
  voltage_reference : Subsystem
  voltage_source : Subsystem
  Vma : Outport
  Vmb : Outport  Port=2
  Vmc : Outport  Port=3
  wires:
  phase_gen/1(grid_emu_phase) -> voltage_reference/1(grid_emu_phase)  "grid_emu_phase"
  voltage_source/2(vn_xi) -> voltage_reference/3(Vxi_n)
  voltage_source/1(vp_xi) -> voltage_reference/2(Vxi_p)
  voltage_source/3(vn_eta) -> voltage_reference/4(Veta_n)
  voltage_reference/3(V3_ref) -> Vmc/1
  voltage_reference/1(V1_ref) -> Vma/1
  voltage_reference/2(V2_ref) -> Vmb/1

== system dual_thyristor_bridge_rectifier/grid/grid_emulator/threephase_vi_measures ==
  Bus Creator : BusCreator  Inputs=6
  Current Sensor : fl_lib/Electrical/Electrical Sensors/Current Sensor
  Current Sensor1 : fl_lib/Electrical/Electrical Sensors/Current Sensor
  Current Sensor2 : fl_lib/Electrical/Electrical Sensors/Current Sensor
  Electrical Reference1 : fl_lib/Electrical/Electrical Elements/Electrical Reference
  Voltage Sensor : fl_lib/Electrical/Electrical Sensors/Voltage Sensor
  Voltage Sensor1 : fl_lib/Electrical/Electrical Sensors/Voltage Sensor
  Voltage Sensor2 : fl_lib/Electrical/Electrical Sensors/Voltage Sensor
  i : Selector  InputPortWidth=6  IndexOptions=Index vector (dialog)  Indices=[4 5 6]  OutputSizes=1
  i_line_abc/u_line_abc : Scope  NumInputPorts=2
      settings: SampleTime=tc  ActiveDisplayYMinimum=-3717.47764  ActiveDisplayYMaximum=2553.67495  DataLoggingVariableName=ScopeData2
  ia_grid : nesl_utility/PS-Simulink Converter  PhysicalDomain=network_engine_domain  SubClassName=ps_output  LeftPortType=input  RightPortType=output  PseudoPeriodic=off  Frequencies=[]  VectorFormat=1-D array  Unit=A  AffineConversion=off
  ib_grid : nesl_utility/PS-Simulink Converter  PhysicalDomain=network_engine_domain  SubClassName=ps_output  LeftPortType=input  RightPortType=output  PseudoPeriodic=off  Frequencies=[]  VectorFormat=1-D array  Unit=A  AffineConversion=off
  ic_grid : nesl_utility/PS-Simulink Converter  PhysicalDomain=network_engine_domain  SubClassName=ps_output  LeftPortType=input  RightPortType=output  PseudoPeriodic=off  Frequencies=[]  VectorFormat=1-D array  Unit=A  AffineConversion=off
  u : Selector  InputPortWidth=6  IndexOptions=Index vector (dialog)  Indices=[1 2 3]  OutputSizes=1
  ua_grid : nesl_utility/PS-Simulink Converter  PhysicalDomain=network_engine_domain  SubClassName=ps_output  LeftPortType=input  RightPortType=output  PseudoPeriodic=off  Frequencies=[]  VectorFormat=1-D array  Unit=V  AffineConversion=off
  ub_grid : nesl_utility/PS-Simulink Converter  PhysicalDomain=network_engine_domain  SubClassName=ps_output  LeftPortType=input  RightPortType=output  PseudoPeriodic=off  Frequencies=[]  VectorFormat=1-D array  Unit=V  AffineConversion=off
  uc_grid : nesl_utility/PS-Simulink Converter  PhysicalDomain=network_engine_domain  SubClassName=ps_output  LeftPortType=input  RightPortType=output  PseudoPeriodic=off  Frequencies=[]  VectorFormat=1-D array  Unit=V  AffineConversion=off
  Ua : PMIOPort  Side=Left
  ua : PMIOPort  Port=2  Side=Right
  Ub : PMIOPort  Port=3  Side=Left
  ub : PMIOPort  Port=4  Side=Right
  Uc : PMIOPort  Port=5  Side=Left
  uc : PMIOPort  Port=6  Side=Right
  wires:
  Bus Creator/1 -> i/1, u/1  "vi_data"
  ib_grid/1 -> Bus Creator/5  "ib"
  ia_grid/1 -> Bus Creator/4  "ia"
  ic_grid/1 -> Bus Creator/6  "ic"
  ua_grid/1 -> Bus Creator/1  "ua"
  ub_grid/1 -> Bus Creator/2  "ub"
  uc_grid/1 -> Bus Creator/3  "uc"
  i/1 -> i_line_abc/u_line_abc/1
  u/1 -> i_line_abc/u_line_abc/2
  connections:
  Current Sensor1/LConn1 -- Ub/RConn1 -- Voltage Sensor1/LConn1
  Electrical Reference1/LConn1 -- Voltage Sensor/RConn2 -- Voltage Sensor2/RConn2 -- Voltage Sensor1/RConn2
  Voltage Sensor/RConn1 -- ua_grid/LConn1
  Current Sensor/RConn2 -- ua/RConn1
  Voltage Sensor1/RConn1 -- ub_grid/LConn1
  Voltage Sensor2/LConn1 -- Current Sensor2/LConn1 -- Uc/RConn1
  Current Sensor/LConn1 -- Ua/RConn1 -- Voltage Sensor/LConn1
  Current Sensor1/RConn2 -- ub/RConn1
  Voltage Sensor2/RConn1 -- uc_grid/LConn1
  ib_grid/LConn1 -- Current Sensor1/RConn1
  ia_grid/LConn1 -- Current Sensor/RConn1
  ic_grid/LConn1 -- Current Sensor2/RConn1
  Current Sensor2/RConn2 -- uc/RConn1

== system dual_thyristor_bridge_rectifier/grid/instantaneus_power/abc2alphabeta ==
  a : Inport
  b : Inport  Port=2
  c : Inport  Port=3
  Gain1 : Gain  Gain=-1/2
  Gain11 : Gain  Gain=-1/2
  Gain2 : Gain  Gain=0
  Gain3 : Gain  Gain=sqrt(3)/2
  Gain4 : Gain  Gain=-sqrt(3)/2
  Gain8 : Gain  Gain=2/3
  Gain9 : Gain  Gain=2/3
  Sum : Sum  Inputs=+++
  Sum1 : Sum  Inputs=+++
  "alpha " : Outport  VectorParamsAs1DForOutWhenUnconnected=off
  "beta " : Outport  Port=2  VectorParamsAs1DForOutWhenUnconnected=off
  wires:
  Sum1/1 -> Gain9/1
  Gain3/1 -> Sum1/2
  Gain8/1 -> "alpha "/1
  Gain1/1 -> Sum/3
  Gain9/1 -> "beta "/1
  Sum/1 -> Gain8/1
  Gain11/1 -> Sum/2
  b/1 -> Gain3/1, Gain11/1
  a/1 -> Gain2/1, Sum/1
  c/1 -> Gain4/1, Gain1/1
  Gain2/1 -> Sum1/1
  Gain4/1 -> Sum1/3

== system dual_thyristor_bridge_rectifier/grid/instantaneus_power/abc2alphabeta  ==
  a : Inport
  b : Inport  Port=2
  c : Inport  Port=3
  Gain1 : Gain  Gain=-1/2
  Gain11 : Gain  Gain=-1/2
  Gain2 : Gain  Gain=0
  Gain3 : Gain  Gain=sqrt(3)/2
  Gain4 : Gain  Gain=-sqrt(3)/2
  Gain8 : Gain  Gain=2/3
  Gain9 : Gain  Gain=2/3
  Sum : Sum  Inputs=+++
  Sum1 : Sum  Inputs=+++
  "alpha " : Outport  VectorParamsAs1DForOutWhenUnconnected=off
  "beta " : Outport  Port=2  VectorParamsAs1DForOutWhenUnconnected=off
  wires:
  Gain3/1 -> Sum1/2
  Gain8/1 -> "alpha "/1
  c/1 -> Gain1/1, Gain4/1
  Gain9/1 -> "beta "/1
  b/1 -> Gain11/1, Gain3/1
  a/1 -> Sum/1, Gain2/1
  Sum1/1 -> Gain9/1
  Gain11/1 -> Sum/2
  Gain2/1 -> Sum1/1
  Sum/1 -> Gain8/1
  Gain4/1 -> Sum1/3
  Gain1/1 -> Sum/3

== system dual_thyristor_bridge_rectifier/grid/instantaneus_power/mavg_p ==
  In1 : Inport
  Gain : Gain  Gain=n1-1
  Gain1 : Gain  Gain=1/n1
  Sum : Sum  Inputs=|++
  Unit Delay : UnitDelay  SampleTime=ts_ctrl_rect  HasFrameUpgradeWarning=on
  Out1 : Outport  VectorParamsAs1DForOutWhenUnconnected=off
  wires:
  Sum/1 -> Gain1/1
  Unit Delay/1 -> Gain/1
  In1/1 -> Sum/1
  Gain1/1 -> Out1/1, Unit Delay/1
  Gain/1 -> Sum/2

== system dual_thyristor_bridge_rectifier/grid/instantaneus_power/mavg_q ==
  In1 : Inport
  Gain : Gain  Gain=n1-1
  Gain1 : Gain  Gain=1/n1
  Sum : Sum  Inputs=|++
  Unit Delay : UnitDelay  SampleTime=ts_ctrl_rect  HasFrameUpgradeWarning=on
  Out1 : Outport  VectorParamsAs1DForOutWhenUnconnected=off
  wires:
  Gain/1 -> Sum/2
  Gain1/1 -> Unit Delay/1, Out1/1
  In1/1 -> Sum/1
  Unit Delay/1 -> Gain/1
  Sum/1 -> Gain1/1

== system dual_thyristor_bridge_rectifier/grid/instantaneus_power/rms ==
  In1 : Inport
  Gain : Gain  Gain=n10-1
  Gain1 : Gain  Gain=1/n10
  Math Function : Math  Operator=magnitude^2  SignedPower=on
  Sqrt : Sqrt
  Sum : Sum  Inputs=|++
  Unit Delay : UnitDelay  SampleTime=ts_ctrl_rect  HasFrameUpgradeWarning=on
  Out1 : Outport  VectorParamsAs1DForOutWhenUnconnected=off
  wires:
  In1/1 -> Math Function/1
  Sum/1 -> Gain1/1
  Gain1/1 -> Sqrt/1, Unit Delay/1
  Unit Delay/1 -> Gain/1
  Math Function/1 -> Sum/1
  Sqrt/1 -> Out1/1
  Gain/1 -> Sum/2

== system dual_thyristor_bridge_rectifier/grid/instantaneus_power/rms1 ==
  In1 : Inport
  Gain : Gain  Gain=n10-1
  Gain1 : Gain  Gain=1/n10
  Math Function : Math  Operator=magnitude^2  SignedPower=on
  Sqrt : Sqrt
  Sum : Sum  Inputs=|++
  Unit Delay : UnitDelay  SampleTime=ts_ctrl_rect  HasFrameUpgradeWarning=on
  Out1 : Outport  VectorParamsAs1DForOutWhenUnconnected=off
  wires:
  Gain/1 -> Sum/2
  Sqrt/1 -> Out1/1
  Math Function/1 -> Sum/1
  Unit Delay/1 -> Gain/1
  Gain1/1 -> Unit Delay/1, Sqrt/1
  Sum/1 -> Gain1/1
  In1/1 -> Math Function/1

== system dual_thyristor_bridge_rectifier/grid/instantaneus_power/rms2 ==
  In1 : Inport
  Gain : Gain  Gain=n10-1
  Gain1 : Gain  Gain=1/n10
  Math Function : Math  Operator=magnitude^2  SignedPower=on
  Sqrt : Sqrt
  Sum : Sum  Inputs=|++
  Unit Delay : UnitDelay  SampleTime=ts_ctrl_rect  HasFrameUpgradeWarning=on
  Out1 : Outport  VectorParamsAs1DForOutWhenUnconnected=off
  wires:
  In1/1 -> Math Function/1
  Sum/1 -> Gain1/1
  Gain1/1 -> Sqrt/1, Unit Delay/1
  Unit Delay/1 -> Gain/1
  Math Function/1 -> Sum/1
  Sqrt/1 -> Out1/1
  Gain/1 -> Sum/2

== system dual_thyristor_bridge_rectifier/grid/instantaneus_power/rms3 ==
  In1 : Inport
  Gain : Gain  Gain=n10-1
  Gain1 : Gain  Gain=1/n10
  Math Function : Math  Operator=magnitude^2  SignedPower=on
  Sqrt : Sqrt
  Sum : Sum  Inputs=|++
  Unit Delay : UnitDelay  SampleTime=ts_ctrl_rect  HasFrameUpgradeWarning=on
  Out1 : Outport  VectorParamsAs1DForOutWhenUnconnected=off
  wires:
  Gain/1 -> Sum/2
  Sqrt/1 -> Out1/1
  Math Function/1 -> Sum/1
  Unit Delay/1 -> Gain/1
  Gain1/1 -> Unit Delay/1, Sqrt/1
  Sum/1 -> Gain1/1
  In1/1 -> Math Function/1

== system dual_thyristor_bridge_rectifier/grid/instantaneus_power/rms4 ==
  In1 : Inport
  Gain : Gain  Gain=n10-1
  Gain1 : Gain  Gain=1/n10
  Math Function : Math  Operator=magnitude^2  SignedPower=on
  Sqrt : Sqrt
  Sum : Sum  Inputs=|++
  Unit Delay : UnitDelay  SampleTime=ts_ctrl_rect  HasFrameUpgradeWarning=on
  Out1 : Outport  VectorParamsAs1DForOutWhenUnconnected=off
  wires:
  In1/1 -> Math Function/1
  Sum/1 -> Gain1/1
  Gain1/1 -> Sqrt/1, Unit Delay/1
  Unit Delay/1 -> Gain/1
  Math Function/1 -> Sum/1
  Sqrt/1 -> Out1/1
  Gain/1 -> Sum/2

== system dual_thyristor_bridge_rectifier/grid/instantaneus_power/rms5 ==
  In1 : Inport
  Gain : Gain  Gain=n10-1
  Gain1 : Gain  Gain=1/n10
  Math Function : Math  Operator=magnitude^2  SignedPower=on
  Sqrt : Sqrt
  Sum : Sum  Inputs=|++
  Unit Delay : UnitDelay  SampleTime=ts_ctrl_rect  HasFrameUpgradeWarning=on
  Out1 : Outport  VectorParamsAs1DForOutWhenUnconnected=off
  wires:
  Gain/1 -> Sum/2
  Sqrt/1 -> Out1/1
  Math Function/1 -> Sum/1
  Unit Delay/1 -> Gain/1
  Gain1/1 -> Unit Delay/1, Sqrt/1
  Sum/1 -> Gain1/1
  In1/1 -> Math Function/1

== system dual_thyristor_bridge_rectifier/load_and_control/controller/pi_voltage_ctrl ==
  vout_ref : Inport
  vout : Inport  Port=2
  1/Ti : Gain  Gain=kp_u_ctrl  SaturateOnIntegerOverflow=on  OutDataTypeStr=Inherit: Same as input  ParamDataTypeStr=Inherit: Same as input
  1/Ti1 : Gain  Gain=180/pi  SaturateOnIntegerOverflow=on  OutDataTypeStr=Inherit: Same as input  ParamDataTypeStr=Inherit: Same as input
  1/Ti2 : Gain  Gain=1/Vdc_traction_normalization_factor  SaturateOnIntegerOverflow=on  OutDataTypeStr=Inherit: Same as input  ParamDataTypeStr=Inherit: Same as input
  Saturation : Saturate  UpperLimit=pi-0.1  LowerLimit=0.1
  Saturation1 : Saturate  UpperLimit=1  LowerLimit=-1
  Sum1 : Sum  Inputs=+++  SaturateOnIntegerOverflow=on
  Sum2 : Sum  Inputs=+-  SaturateOnIntegerOverflow=on
  Sum3 : Sum  Inputs=-+  SaturateOnIntegerOverflow=on
  Trigonometric Function : Trigonometry  Operator=acos
  Unit Delay1 : UnitDelay  SampleTime=ts_ctrl_rect  HasFrameUpgradeWarning=on
  Unit Delay4 : UnitDelay  SampleTime=ts_ctrl_rect  HasFrameUpgradeWarning=on
  Zero-Order Hold1 : ZeroOrderHold  SampleTime=ts_ctrl_rect
  Zero-Order Hold2 : ZeroOrderHold  SampleTime=ts_ctrl_rect
  kp : Gain  Gain=ki_u_ctrl*ts_ctrl_rect  SaturateOnIntegerOverflow=on  OutDataTypeStr=Inherit: Same as input  ParamDataTypeStr=Inherit: Same as input
  w : Outport  VectorParamsAs1DForOutWhenUnconnected=off
  wires:
  Saturation1/1 -> Trigonometric Function/1, Sum3/2
  Unit Delay1/1 -> w/1
  1/Ti2/1 -> Zero-Order Hold2/1
  vout_ref/1 -> Zero-Order Hold1/1
  vout/1 -> 1/Ti2/1
  Saturation/1 -> Unit Delay1/1
  Sum3/1 -> Unit Delay4/1
  1/Ti/1 -> Sum1/1, Sum3/1
  Zero-Order Hold1/1 -> Sum2/1
  Zero-Order Hold2/1 -> Sum2/2
  Trigonometric Function/1 -> Saturation/1
  Unit Delay4/1 -> Sum1/3
  Sum1/1 -> Saturation1/1
  Sum2/1 -> 1/Ti/1, kp/1
  kp/1 -> Sum1/2

== system dual_thyristor_bridge_rectifier/dual_rectifier_bridge/neg_bridge/firing1/oscillator ==
  Data Type Conversion : DataTypeConversion  OutDataTypeStr=double  SaturateOnIntegerOverflow=off  RndMeth=Floor
  Logical Operator1 : Logic  Operator=NOT  AllPortsSameDT=off  OutDataTypeStr=boolean
  Rate Transition : RateTransition  OutPortSampleTime=ts
  Simulink-PS Converter : nesl_utility/Simulink-PS Converter  PhysicalDomain=network_engine_domain  SubClassName=ps_input  LeftPortType=input  RightPortType=output  PseudoPeriodic=off  Frequencies=[]  NoiseDistribution=none  NoiseParameters=[]  Unit=1  AffineConversion=off  FilteringAndDerivatives=provide  SimscapeFilterOrder=1  InputFilterTimeConstant=0.001  UdotUserProvided=0
  Unit Delay1 : UnitDelay  SampleTime=Tcontrol_rect  HasFrameUpgradeWarning=on
  output : PMIOPort  Side=Right
  wires:
  Data Type Conversion/1 -> Rate Transition/1
  Unit Delay1/1 -> Logical Operator1/1
  Logical Operator1/1 -> Unit Delay1/1, Data Type Conversion/1
  Rate Transition/1 -> Simulink-PS Converter/1
  connections:
  Simulink-PS Converter/RConn1 -- output/RConn1

== system dual_thyristor_bridge_rectifier/dual_rectifier_bridge/neg_bridge/firing2/oscillator ==
  Data Type Conversion : DataTypeConversion  OutDataTypeStr=double  SaturateOnIntegerOverflow=off  RndMeth=Floor
  Logical Operator1 : Logic  Operator=NOT  AllPortsSameDT=off  OutDataTypeStr=boolean
  Rate Transition : RateTransition  OutPortSampleTime=ts
  Simulink-PS Converter : nesl_utility/Simulink-PS Converter  PhysicalDomain=network_engine_domain  SubClassName=ps_input  LeftPortType=input  RightPortType=output  PseudoPeriodic=off  Frequencies=[]  NoiseDistribution=none  NoiseParameters=[]  Unit=1  AffineConversion=off  FilteringAndDerivatives=provide  SimscapeFilterOrder=1  InputFilterTimeConstant=0.001  UdotUserProvided=0
  Unit Delay1 : UnitDelay  SampleTime=Tcontrol_rect  HasFrameUpgradeWarning=on
  output : PMIOPort  Side=Right
  wires:
  Logical Operator1/1 -> Data Type Conversion/1, Unit Delay1/1
  Unit Delay1/1 -> Logical Operator1/1
  Data Type Conversion/1 -> Rate Transition/1
  Rate Transition/1 -> Simulink-PS Converter/1
  connections:
  Simulink-PS Converter/RConn1 -- output/RConn1
